simulink model "Wind_Turbine"  (R2025a)
settings: Solver=ode23t  StartTime=0.0  StopTime=70  MaxStep=0.01  RelTol=1e-4  AbsTol=1e-4  EnableMultiTasking=on
PreLoadFcn:
  | warning off Simulink:Commands:LoadMdlParameterizedLink
PostLoadFcn:
  | warning off Simulink:blocks:MatchingGotoNotFound
  | warning off Simulink:blocks:MatchingFromNotFound
  | warning('off','Simulink:SL_OutputNotConnected');
  | warning off Simulink:Engine:SaveWithParameterizedLinks_Warning
  | warning off Simulink:Engine:SaveWithDisabledLinks_Warning
  | warning('off','Simulink:fixpoint:fxpParameterPrecisionLoss');
  | warning off Simulink:blocks:DTConversionUncessary
  | warning off ne_sli:simulator:input:FilteredInputs
  | warning off MATLAB:nearlySingularMatrix
  | 
  | warning off xPCTarget:modeloptions:StackIncrease
  | warning off xPCTarget:sampleTime:sampleTimeInvariance
  | warning off Simulink:blocks:TDelayFixedBuffer
  | 
  | Setup_WT_Configurations
StartFcn:
  | tic
StopFcn:
  | Elapsed_Sim_Time = toc;
  | disp(['Elapsed time is ' num2str(Elapsed_Sim_Time)]);
undefined symbols (not defined in the file): sigbuilder_block, WT_Params, X, Y, Z
libraries: sm_lib x6, Wind_Lib x4, Yaw_System_Lib x4, Generator_Lib x3, Pitch_System_Lib x3, Pitch_Controller_Lib x3, Main_Controller_Lib x2, Geartrain_Lib x2, Hub_Axis_Lib x2, nesl_utility x2, Blades_Lib x1, Tower x1
Description:
  | Copyright 2009-2025 The MathWorks, Inc. MathWorks, Inc.
settings Model: ExtModeTrigDuration=100  Creator=smiller  LastModifiedBy=smiller
settings SolverCC: AutoScaleAbsTol=off  MaxConsecutiveMinStep=5  AlgebraicLoopSolver=TrustRegion  PositivePriorityOrder=on
settings DataIOCC: SaveFinalState=on  SaveFormat=StructureWithTime  ReturnWorkspaceOutputs=off
settings OptimizationCC: BlockReduction=off  OptimizeBlockIOStorage=off  BufferReuse=off  ReuseModelBlockBuffer=off  GlobalBufferReuse=off  ExpressionFolding=off  ExpressionDepthLimit=2147483647.0  LocalBlockOutputs=off  ZeroExternalMemoryAtStartup=off  ZeroInternalMemoryAtStartup=off  OptimizeDataStoreBuffers=off  BusAssignmentInplaceUpdate=off
settings DebuggingCC: AlgebraicLoopMsg=error  ArtificialAlgebraicLoopMsg=none  UnderspecifiedInitializationDetection=Classic  MergeDetectMultiDrivingBlocksExec=none  Int32ToFloatConvMsg=none  UnnecessaryDatatypeConvMsg=warning  FcnCallInpInsideContextMsg=warning  UnconnectedInputMsg=warning  UnconnectedOutputMsg=warning  UnconnectedLineMsg=warning  AllowSymbolicDim=off  StateNameClashWarn=warning  PregeneratedLibrarySubsystemCodeDiagnostic=none  SFUnexpectedBacktrackingDiag=warning  SFNoUnconditionalDefaultTransitionDiag=warning  SFExecutionAtInitializationDiag=none  ArithmeticOperatorsInVariantConditions=warning
settings HardwareCC: TargetBitPerPointer=64.0  TargetBitPerSizeT=64.0  TargetBitPerPtrDiffT=64.0  TargetLongLongMode=on  TargetIntDivRoundTo=Zero  TargetEndianess=LittleEndian  TargetWordSize=64.0  TargetHWDeviceType=MATLAB Host
settings ModelReferenceCC: EnableRefExpFcnMdlSchedulingChecks=on  PropagateSignalLabelsOutOfModel=off
settings SFSimCC: SimUseLocalCustomCode=off  SimParseCustomCode=off  CustomCodeUndefinedFunction=UseInterfaceOnly
settings RTWCC: RTWUseLocalCustomCode=off  Toolchain=Simulink Real-Time Toolchain  BuildConfiguration=Faster Runs  TargetLang=C++  GPUComputeCapability=3.5  DLArmComputeVersion=19.05
settings CodeAppCC: StateflowObjectComments=on
settings GRTTargetCC: TargetLangStandard=C++03 (ISO)  CodeInterfacePackaging=C++ class
settings ConfigComp: CovMetricSettings=dw  CovSaveCumulativeToWorkspaceVar=on  CovSaveSingleToWorkspaceVar=on  CovExternalEMLEnable=off  CovSFcnEnable=off
settings SimscapeCC: ExplicitSolverDiagnosticOptions=none  SimscapeNormalizeSystem=off  SimscapeLogType=all  SimscapeLogName=simlog_Wind_Turbine  SimscapeLogLimitData=off
settings ConfigurationSet: Description=SimMechanics 2G
settings ExplorerConfigSet: InternalSimMechanicsExplorerSettings="<ExplorerConfiguration><canonicalview>default</canonicalview><TilePanel><TileInfo><Tiles Columns=\"2\" Count=\"3\" Rows=\"2\"><Column Left=\"2\" Weight=\"0.6616\"/><Column Left=\"1076\" Weight=\"0.3384\"/><Column Left=\"1628\"/><Row Top=\"2\" Weight=\"0.4995\"/><Row Top=\"507\" Weight=\"0.5005\"/><Row Top=\"1014\"/><Tile Height=\"1\" Width=\"1\" X=\"0\" Y=\"0\"/><Tile Height=\"1\" Width=\"1\" X=\"0\" Y=\"1\"/><Tile Height=\"2\" Width=\"1\" X=\"1\" Y=\"0\"/></Tiles></TileInfo><SceneInfo><SceneViewer><BGColor><R>0.80000001192092896</R><G>1</G><B>1</B></BGColor><Camera><Position><X>151.73049973570119</X><Y>118.34405364859263</Y><Z>134.40663706667596</Z></Position><Center><X>-10.795458452286731</X><Y>-8.3649508446642677</Y><Z>101.0263657071233</Z></Center><Up><X>-0.12932527544138767</X><Y>-0.094165770600414006</Y><Z>0.98712095549595125</Z></Up><Left>-10.158594940113018</Left><Right>10.158594940113018</Right><Bottom>-7.1278539082560997</Bottom><Top>7.1278539082560997</Top></Camera></SceneViewer><SceneViewer><BGColor><R>0.80000001192092896</R><G>1</G><B>1</B></BGColor><Camera><Position><X>3.5719318734898633</X><Y>-0.12848459366052295</Y><Z>225.51131574619058</Z></Position><Center><X>-2.4920494569662206</X><Y>-0.0648600322177105</Y><Z>66.260519833710546</Z></Center><Up><X>0.0026243051834802709</X><Y>-0.99999643177881292</Y><Z>-0.00049945164542893202</Z></Up><Left>-11.826399210226041</Left><Right>11.826399210226041</Right><Bottom>-5.4233487502515896</Bottom><Top>5.4233487502515896</Top></Camera></SceneViewer><SceneViewer><BGColor><R>0.80000001192092896</R><G>1</G><B>1</B></BGColor><Camera><Position><X>121.9852231624925</X><Y>91.296071561311123</Y><Z>95.392428744838412</Z></Position><Center><X>2.8343002263369788</X><Y>-1.5967499794196209</Y><Z>70.920706290818515</Z></Center><Up><X>-0.12932527544138767</X><Y>-0.094165770600414006</Y><Z>0.98712095549595125</Z></Up><Left>-36.268603134155278</Left><Right>36.268603134155278</Right><Bottom>-73.406224822998055</Bottom><Top>73.406224822998055</Top></Camera></SceneViewer></SceneInfo></TilePanel></ExplorerConfiguration>"

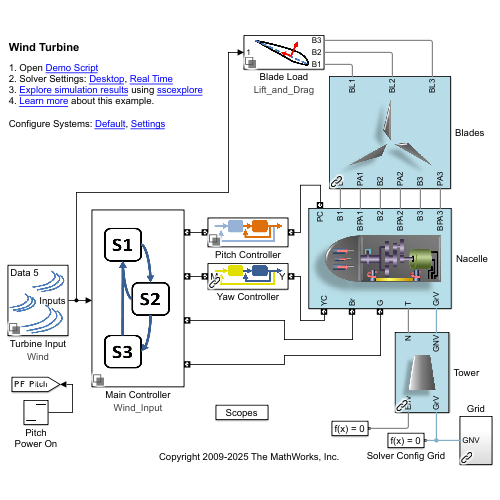
[thumbnail: Simulink's stored preview of the top-level diagram]
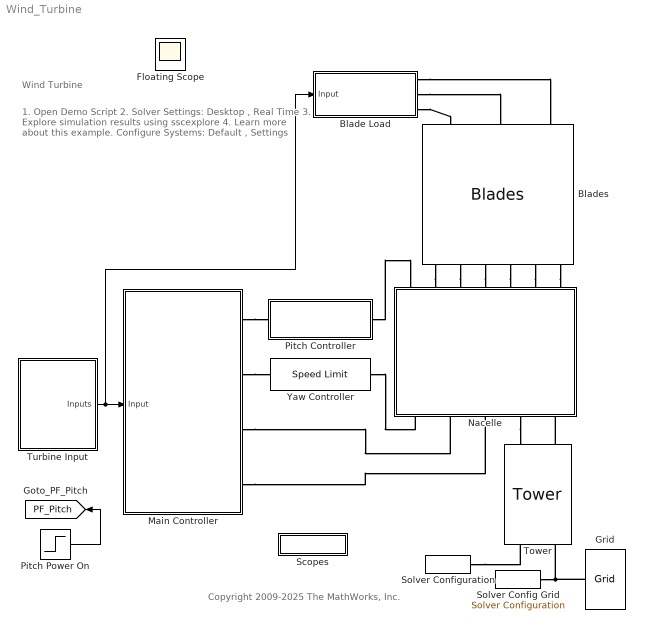
== system Wind_Turbine ==
  note: Copyright 2009-2025 The MathWorks, Inc.
  note: 1. Open Demo Script
      | 2. Solver Settings: Desktop , Real Time
      | 3. Explore simulation results using sscexplore
      | 4. Learn more about this example.
      |
      | Configure Systems: Default , Settings
  note: Wind Turbine
  Blade Load : Subsystem  Variant=on  VariantControlMode=label  LabelModeActiveChoice=Lift_and_Drag
      settings: AttributesFormatString=%<ActiveVariant>
      mask Display:
      | blk = wind_turbine_activeVariantBlock(gcb);
      | eval(get_param(blk, 'MaskDisplay'));
  Blades : Blades_Lib/Blades  RequirementInfo={} %GIDa_b4b772d6_2a4e_4d26_8c7e_f4f3f2f69a80  SystemSampleTime=-1  VariantActivationTime=update diagram  EmptyChoice=off  PassThrough=off  PassThroughVariantControl=(default)  EmptyChoiceVariantControl=(default)  AllowFlexibleInterface=on  Latency=0  AutoFrameSizeCalculation=off
  Grid : Generator_Lib/Grid  SystemSampleTime=-1  VariantActivationTime=update diagram  EmptyChoice=off  PassThrough=off  PassThroughVariantControl=(default)  EmptyChoiceVariantControl=(default)  AllowFlexibleInterface=on  Latency=0  AutoFrameSizeCalculation=off
  Main Controller : Subsystem  RequirementInfo={} %GIDa_306d441f_b8e1_436d_a194_501ebadfbc9d  Variant=on  VariantControlMode=label  LabelModeActiveChoice=Wind_Input
      settings: AttributesFormatString=%<ActiveVariant>
      mask Display:
      | blk = wind_turbine_activeVariantBlock(gcb);
      | eval(get_param(blk, 'MaskDisplay'));
  Nacelle : Subsystem
      mask Display:
      | PiA_Char = get_param([bdroot '/Nacelle/Pitch System'],'ActiveVariant');
      | YaA_Char = get_param([bdroot '/Nacelle/Yaw System'],'ActiveVariant');
      | Hub_Char = get_param([bdroot '/Nacelle/Hub Axis'],'ActiveVariant');
      | Gea_Char = get_param([bdroot '/Nacelle/Geartrain'],'ActiveVariant');
      | Gen_Char = get_param([bdroot '/Nacelle/Generator'],'ActiveVariant');
      | 
      | if(length(YaA_Char)<7)
      |     YaA_Char = 'LockedL';
      | end
      | 
      | image_str = ['Pi' PiA_Char(1) 'Ya' upper(YaA_Char(7)) 'Hu' Hub_Char(1) 'Ge' Gea_Char(1) 'Gn' Gen_Char(1)];
      | try
      |     image(['Nacelle_' image_str '_IMAGE.jpg']);
      | catch
      |     image('Nacelle_IMAGE.jpg');
      | end
  Pitch Power On : Step  Time=20  Before=24  After=24  SampleTime=0
  Pitch Controller : Subsystem  Variant=on  VariantControlMode=label  LabelModeActiveChoice=PI_on_AoA
      settings: AttributesFormatString=%<ActiveVariant>
      mask Display:
      | blk = wind_turbine_activeVariantBlock(gcb);
      | eval(get_param(blk, 'MaskDisplay'));
  Scopes : Subsystem
      mask Display: disp('Scopes');
  Solver Configuration : nesl_utility/Solver Configuration  PhysicalDomain=network_engine_domain  SubClassName=solver  LeftPortType=input  RightPortType=generic  Tones=[]  Harmonics=[]  SimulateNoise=off  Profile=off  UseLocalSampling=off  EnableSwitchedLinearOptims=on  FrequencyDomain=off  UseCCode=off  RelTol=0.001  AbsTol=1e-06  MinStep=1e-09  ToWorkspace=off  RevertToSquareIcSolve=off  NumHomotopyIterations=100  PhasorMode=off  PhasorModeNumHarmonics=1  ConsistencySolver=NEWTON_FTOL  IndexReductionMethod=DerivativeReplacement  DoDC=off  ResidualTolerance=1e-9  ConsistencyTolSource=GLOBAL  ConsistencyAbsTol=0.001  ConsistencyRelTol=0.001  ConsistencyTolFactor=0.001  UseLocalSolver=off  LocalSolverChoice=NE_BACKWARD_EULER_ADVANCER  ResolveIndetEquations=on  FunctionEvalNumThread=1  LocalSolverSampleTime=0.01  DoFixedCost=off  MaxNonlinIter=3  MaxModeIter=2  ComputeImpulses=off  ImpulseIterations=2  LinearAlgebra=Sparse  LinearAlgebraNumThread=0  EquationFormulation=NE_TIME_EF  DelaysMemoryBudget=1024  AutomaticFiltering=on  FilteringTimeConstant=0.001  PartitionStorageMethod=AS_NEEDED  PartitionMemoryBudget=1024  PartitionMethod=FAST  MultibodyUseLocalSolver=off  MultibodyLocalSolverChoice=ODE1  MultibodyLocalSolverSampleTime=0.001
  Solver Config Grid : nesl_utility/Solver Configuration  PhysicalDomain=network_engine_domain  SubClassName=solver  LeftPortType=input  RightPortType=generic  Tones=[]  Harmonics=[]  SimulateNoise=off  Profile=off  UseLocalSampling=off  EnableSwitchedLinearOptims=on  FrequencyDomain=off  UseCCode=off  RelTol=0.001  AbsTol=0.001  MinStep=1e-09  ToWorkspace=off  RevertToSquareIcSolve=off  NumHomotopyIterations=100  PhasorMode=off  PhasorModeNumHarmonics=1  ConsistencySolver=NEWTON_XTOL_AFTER_FTOL  IndexReductionMethod=None  DoDC=off  ResidualTolerance=1e-09  ConsistencyTolSource=GLOBAL  ConsistencyAbsTol=0.001  ConsistencyRelTol=0.001  ConsistencyTolFactor=1  UseLocalSolver=off  LocalSolverChoice=NE_BACKWARD_EULER_ADVANCER  ResolveIndetEquations=off  FunctionEvalNumThread=1  LocalSolverSampleTime=5e-5  DoFixedCost=off  MaxNonlinIter=2  MaxModeIter=2  ComputeImpulses=off  ImpulseIterations=2  LinearAlgebra=auto  LinearAlgebraNumThread=0  EquationFormulation=NE_FREQUENCY_TIME_EF  DelaysMemoryBudget=1024  AutomaticFiltering=off  FilteringTimeConstant=0.001  PartitionStorageMethod=AS_NEEDED  PartitionMemoryBudget=1024  PartitionMethod=ROBUST  MultibodyUseLocalSolver=off  MultibodyLocalSolverChoice=ODE1  MultibodyLocalSolverSampleTime=0.001
  Tower : Tower/Tower  RequirementInfo={} %GIDa_4943b1c2_7ab1_472c_939d_e8be874b5a74  SystemSampleTime=-1  VariantActivationTime=update diagram  EmptyChoice=off  PassThrough=off  PassThroughVariantControl=(default)  EmptyChoiceVariantControl=(default)  AllowFlexibleInterface=on  Latency=0  AutoFrameSizeCalculation=off
  Turbine Input : Subsystem  Variant=on  VariantControlMode=label  LabelModeActiveChoice=Wind
      settings: AttributesFormatString=%<ActiveVariant>
      mask Display:
      | blk = wind_turbine_activeVariantBlock(gcb);
      | eval(get_param(blk, 'MaskDisplay'));
      | 
      | 
      | if strcmp(get_param(gcb,'activevariant'),'Wind')
      |     [gr_ind, l] = signalbuilder([gcb '/Wind/Wind Input'], 'activegroup');
      |     text(0.05,0.9,['Data ' num2str(gr_ind)]);
      | end
  Yaw Controller : Yaw_Controller_Lib/Speed Limit  SystemSampleTime=-1  VariantActivationTime=update diagram  EmptyChoice=off  PassThrough=off  PassThroughVariantControl=(default)  EmptyChoiceVariantControl=(default)  AllowFlexibleInterface=on  Latency=0  AutoFrameSizeCalculation=off
  Floating Scope : Scope
  tag scope: PF_Pitch=global
  wires:
  Pitch Power On/1 -> [PF_Pitch]
  Turbine Input/1(Inputs) -> Main Controller/1(Input), Blade Load/1(Input)
  connections:
  Blades/LConn1 -- Nacelle/LConn2
  Pitch Controller/RConn1 -- Nacelle/LConn1
  Main Controller/RConn1 -- Pitch Controller/LConn1
  Nacelle/RConn4 -- Tower/LConn1
  Solver Configuration/RConn1 -- Tower/RConn1
  Blades/LConn5 -- Nacelle/LConn6
  Blades/LConn4 -- Nacelle/LConn5
  Blades/LConn3 -- Nacelle/LConn4
  Blades/LConn2 -- Nacelle/LConn3
  Blades/LConn6 -- Nacelle/LConn7
  Main Controller/RConn2 -- Yaw Controller/LConn1
  Main Controller/RConn4 -- Nacelle/RConn3
  Main Controller/RConn3 -- Nacelle/RConn2
  Blade Load/RConn3 -- Blades/RConn1
  Blade Load/RConn2 -- Blades/RConn2
  Blade Load/RConn1 -- Blades/RConn3
  Yaw Controller/RConn1 -- Nacelle/RConn1
  Solver Config Grid/RConn1 -- Grid/RConn1 -- Tower/RConn2
  Tower/LConn2 -- Nacelle/RConn5

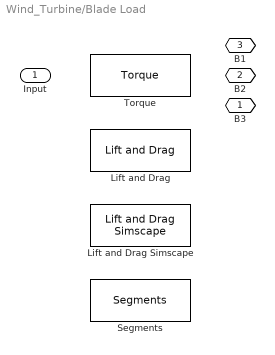
== system Wind_Turbine/Blade Load ==
  Input : Inport
  Lift and Drag : Wind_Lib/Lift and Drag  SystemSampleTime=-1  VariantControl=Lift_and_Drag  VariantActivationTime=update diagram  EmptyChoice=off  PassThrough=off  PassThroughVariantControl=(default)  EmptyChoiceVariantControl=(default)  AllowFlexibleInterface=on  Latency=0  AutoFrameSizeCalculation=off
  Lift and Drag Simscape : Wind_Lib/Lift and Drag Simscape  SystemSampleTime=-1  VariantControl=Lift_and_Drag_Simscape  VariantActivationTime=update diagram  EmptyChoice=off  PassThrough=off  PassThroughVariantControl=(default)  EmptyChoiceVariantControl=(default)  AllowFlexibleInterface=on  Latency=0  AutoFrameSizeCalculation=off
  Segments : Wind_Lib/Segments  SystemSampleTime=-1  VariantControl=Segments  VariantActivationTime=update diagram  EmptyChoice=off  PassThrough=off  PassThroughVariantControl=(default)  EmptyChoiceVariantControl=(default)  AllowFlexibleInterface=on  Latency=0  AutoFrameSizeCalculation=off
  Torque : Wind_Lib/Torque  SystemSampleTime=-1  VariantControl=Torque  VariantActivationTime=update diagram  EmptyChoice=off  PassThrough=off  PassThroughVariantControl=(default)  EmptyChoiceVariantControl=(default)  AllowFlexibleInterface=on  Latency=0  AutoFrameSizeCalculation=off
  B3 : PMIOPort  Side=Right
  B2 : PMIOPort  Port=2  Side=Right
  B1 : PMIOPort  Port=3  Side=Right

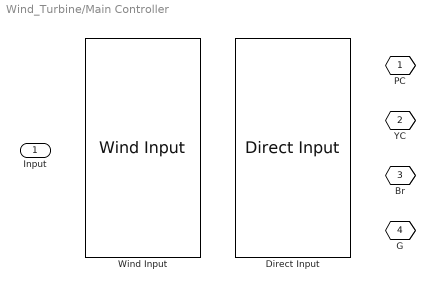
== system Wind_Turbine/Main Controller ==
  Input : Inport
  Direct Input : Main_Controller_Lib/Direct Input  SystemSampleTime=-1  VariantControl=Direct_Input  VariantActivationTime=update diagram  EmptyChoice=off  PassThrough=off  PassThroughVariantControl=(default)  EmptyChoiceVariantControl=(default)  AllowFlexibleInterface=on  Latency=0  AutoFrameSizeCalculation=off
  Wind Input : Main_Controller_Lib/Wind Input  SystemSampleTime=-1  VariantControl=Wind_Input  VariantActivationTime=update diagram  EmptyChoice=off  PassThrough=off  PassThroughVariantControl=(default)  EmptyChoiceVariantControl=(default)  AllowFlexibleInterface=on  Latency=0  AutoFrameSizeCalculation=off
  PC : PMIOPort  Tag=PMCPort  Side=Right
  YC : PMIOPort  Tag=PMCPort  Port=2  Side=Right
  Br : PMIOPort  Tag=PMCPort  Port=3  Side=Right
  G : PMIOPort  Tag=PMCPort  Port=4  Side=Right

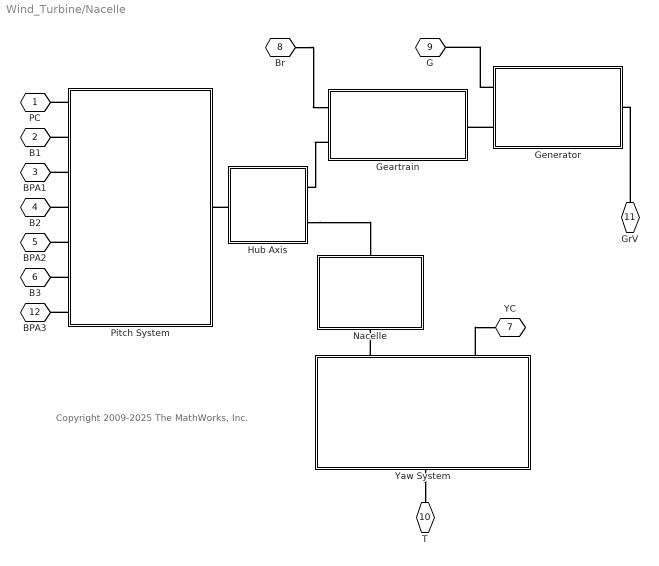
== system Wind_Turbine/Nacelle ==
  note: Copyright 2009-2025 The MathWorks, Inc.
  Geartrain : Subsystem  RequirementInfo={} %GIDa_0de6bbf9_bd2a_4f23_951e_791819310b87  Variant=on  VariantControlMode=label  LabelModeActiveChoice=Ideal
      settings: AttributesFormatString=%<ActiveVariant>
      mask Display:
      | blk = wind_turbine_activeVariantBlock(gcb);
      | eval(get_param(blk, 'MaskDisplay'));
  Generator : Subsystem  Variant=on  VariantControlMode=label  LabelModeActiveChoice=Full
      settings: AttributesFormatString=%<ActiveVariant>
      mask Display:
      | blk = wind_turbine_activeVariantBlock(gcb);
      | eval(get_param(blk, 'MaskDisplay'));
  Hub Axis : Subsystem  Tag=CustomStyle  Variant=on  VariantControlMode=label  LabelModeActiveChoice=Rotate
      settings: AttributesFormatString=%<ActiveVariant>
      mask Display:
      | blk = wind_turbine_activeVariantBlock(gcb);
      | eval(get_param(blk, 'MaskDisplay'));
  Nacelle : Subsystem
      mask Display:
      | image('Nacelle_Housing_IMAGE.jpg');
      | port_label('RConn',1,'N');
      | port_label('LConn',1,'YR');
  Pitch System : Subsystem  Tag=CustomStyle  RequirementInfo={} %GIDa_c1f640a7_49b6_45bd_a761_32e6bbcf8fa3  Variant=on  VariantControlMode=label  LabelModeActiveChoice=Ideal
      settings: AttributesFormatString=%<ActiveVariant>
      mask Display:
      | blk = wind_turbine_activeVariantBlock(gcb);
      | eval(get_param(blk, 'MaskDisplay'));
  Yaw System : Subsystem  Tag=CustomStyle  RequirementInfo={} %GIDa_39d3e21d_5d00_42ae_be4b_0d3d8be28763  Variant=on  VariantControlMode=label  LabelModeActiveChoice=Ideal_Actuator
      settings: AttributesFormatString=%<ActiveVariant>
      mask Display:
      | blk = wind_turbine_activeVariantBlock(gcb);
      | eval(get_param(blk, 'MaskDisplay'));
  PC : PMIOPort  Tag=PMCPort  Side=Left
  B1 : PMIOPort  Tag=PMCPort  Port=2  Side=Left
  BPA1 : PMIOPort  Tag=PMCPort  Port=3  Side=Left
  B2 : PMIOPort  Tag=PMCPort  Port=4  Side=Left
  BPA2 : PMIOPort  Tag=PMCPort  Port=5  Side=Left
  B3 : PMIOPort  Tag=PMCPort  Port=6  Side=Left
  YC : PMIOPort  Tag=PMCPort  Port=7  Side=Right
  Br : PMIOPort  Tag=PMCPort  Port=8  Side=Right
  G : PMIOPort  Tag=PMCPort  Port=9  Side=Right
  T : PMIOPort  Tag=PMCPort  Port=10  Side=Right
  GrV : PMIOPort  Tag=PMCPort  Port=11  Side=Right
  BPA3 : PMIOPort  Tag=PMCPort  Port=12  Side=Left
  connections:
  Hub Axis/LConn1 -- Pitch System/RConn1
  Yaw System/RConn1 -- Nacelle/LConn1
  Yaw System/LConn1 -- T/RConn1
  Br/RConn1 -- Geartrain/LConn1
  Pitch System/LConn7 -- BPA3/RConn1
  Pitch System/LConn5 -- BPA2/RConn1
  Pitch System/LConn3 -- BPA1/RConn1
  Pitch System/LConn6 -- B3/RConn1
  Generator/LConn2 -- Geartrain/RConn1
  Generator/LConn1 -- G/RConn1
  Pitch System/LConn1 -- PC/RConn1
  Pitch System/LConn4 -- B2/RConn1
  Pitch System/LConn2 -- B1/RConn1
  Hub Axis/RConn2 -- Nacelle/RConn1
  Yaw System/RConn2 -- YC/RConn1
  Geartrain/LConn2 -- Hub Axis/RConn1
  GrV/RConn1 -- Generator/RConn1

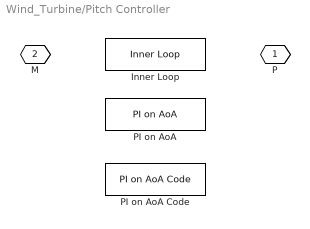
== system Wind_Turbine/Pitch Controller ==
  Inner Loop : Pitch_Controller_Lib/Inner Loop  SystemSampleTime=-1  VariantControl=Inner_Loop  VariantActivationTime=update diagram  EmptyChoice=off  PassThrough=off  PassThroughVariantControl=(default)  EmptyChoiceVariantControl=(default)  AllowFlexibleInterface=on  Latency=0  AutoFrameSizeCalculation=off
  PI on AoA : Pitch_Controller_Lib/PI on AoA  SystemSampleTime=-1  VariantControl=PI_on_AoA  VariantActivationTime=update diagram  EmptyChoice=off  PassThrough=off  PassThroughVariantControl=(default)  EmptyChoiceVariantControl=(default)  AllowFlexibleInterface=on  Latency=0  AutoFrameSizeCalculation=off
  PI on AoA Code : Pitch_Controller_Lib/PI on AoA Code  SystemSampleTime=-1  VariantControl=PI_on_AoA_Code  VariantActivationTime=update diagram  EmptyChoice=off  PassThrough=off  PassThroughVariantControl=(default)  EmptyChoiceVariantControl=(default)  AllowFlexibleInterface=on  Latency=0  AutoFrameSizeCalculation=off
  P : PMIOPort  Tag=PMCPort  Side=Right
  M : PMIOPort  Tag=PMCPort  Port=2  Side=Left

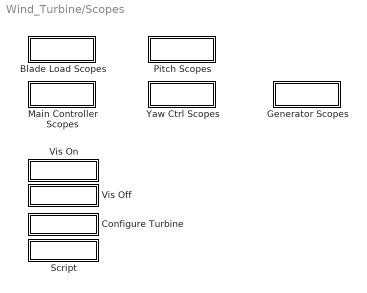
== system Wind_Turbine/Scopes ==
  Blade Load Scopes : Subsystem  ReferencedSubsystem=Blade_Load_Scopes
  Configure Turbine : Subsystem
      mask Display: disp('Configs');
  Generator Scopes : Subsystem  ReferencedSubsystem=Generator_Scopes
  Main Controller Scopes : Subsystem  ReferencedSubsystem=Main_Controller_Scopes
  Pitch Scopes : Subsystem  ReferencedSubsystem=Pitch_Scopes
  Script : Subsystem
      settings: OpenFcn=open('Wind_Turbine_Demo_Script.html')
      mask Display: disp('Script')
  Vis Off : Subsystem
      settings: OpenFcn=set_param(bdroot,'SimMechanicsOpenEditorOnUpdate','off');
      mask Display: disp('Vis Off')
  Vis On : Subsystem
      settings: OpenFcn=set_param(bdroot,'SimMechanicsOpenEditorOnUpdate','on');
      mask Display: disp('Vis On')
  Yaw Ctrl Scopes : Subsystem  ReferencedSubsystem=Yaw_Scopes

== system Wind_Turbine/Turbine Input ==
  Commands : Subsystem  VariantControl=Commands
      mask Display:
      | image(imread('Turbine_Input_Commands_IMAGE.jpg'));
      | port_label('output',1,'Inputs');
  Wind : Subsystem  VariantControl=Wind
      mask Display:
      | image('Turbine_Input_Wind_IMAGE.jpg');
      | port_label('output',1,'Inputs');
  Inputs : Outport  VectorParamsAs1DForOutWhenUnconnected=off

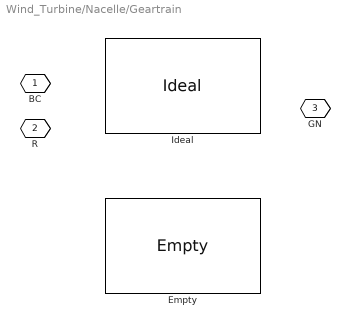
== system Wind_Turbine/Nacelle/Geartrain ==
  Empty : Geartrain_Lib/Empty  SystemSampleTime=-1  VariantControl=Empty  VariantActivationTime=update diagram  EmptyChoice=off  PassThrough=off  PassThroughVariantControl=(default)  EmptyChoiceVariantControl=(default)  AllowFlexibleInterface=on  Latency=0  AutoFrameSizeCalculation=off
  Ideal : Geartrain_Lib/Ideal  SystemSampleTime=-1  VariantControl=Ideal  VariantActivationTime=update diagram  EmptyChoice=off  PassThrough=off  PassThroughVariantControl=(default)  EmptyChoiceVariantControl=(default)  AllowFlexibleInterface=on  Latency=0  AutoFrameSizeCalculation=off
  BC : PMIOPort  Tag=PMCPort  Side=Left
  R : PMIOPort  Tag=PMCPort  Port=2  Side=Left
  GN : PMIOPort  Tag=PMCPort  Port=3  Side=Right

== system Wind_Turbine/Nacelle/Generator ==
  Full : Generator_Lib/Full  SystemSampleTime=-1  VariantControl=Full  VariantActivationTime=update diagram  EmptyChoice=off  PassThrough=off  PassThroughVariantControl=(default)  EmptyChoiceVariantControl=(default)  AllowFlexibleInterface=on  Latency=0  AutoFrameSizeCalculation=off
  Simple : Generator_Lib/Simple  SystemSampleTime=-1  VariantControl=Simple  VariantActivationTime=update diagram  EmptyChoice=off  PassThrough=off  PassThroughVariantControl=(default)  EmptyChoiceVariantControl=(default)  AllowFlexibleInterface=on  Latency=0  AutoFrameSizeCalculation=off
  M : PMIOPort  Tag=PMCPort  Side=Left
  G : PMIOPort  Port=2  Side=Left
  GrV : PMIOPort  Port=3  Side=Right

== system Wind_Turbine/Nacelle/Hub Axis ==
  Locked : Hub_Axis_Lib/Locked  SystemSampleTime=-1  VariantControl=Locked  VariantActivationTime=update diagram  EmptyChoice=off  PassThrough=off  PassThroughVariantControl=(default)  EmptyChoiceVariantControl=(default)  AllowFlexibleInterface=on  Latency=0  AutoFrameSizeCalculation=off
  Rotate : Hub_Axis_Lib/Rotate  SystemSampleTime=-1  VariantControl=Rotate  VariantActivationTime=update diagram  EmptyChoice=off  PassThrough=off  PassThroughVariantControl=(default)  EmptyChoiceVariantControl=(default)  AllowFlexibleInterface=on  Latency=0  AutoFrameSizeCalculation=off
  G : PMIOPort  Side=Right
  R : PMIOPort  Port=2  Side=Left
  N : PMIOPort  Port=3  Side=Right

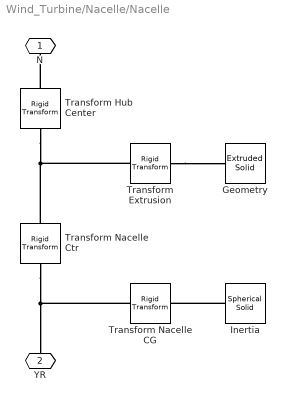
== system Wind_Turbine/Nacelle/Nacelle ==
  Geometry : sm_lib/Body Elements/Extruded Solid  ExtrusionType=General  PolygonNumSides=3  PolygonOuterRadius=1  PolygonOuterRadiusUnits=m  ExportEntireGeometry=off  ExtrusionCrossSection=WT_Params.Nacelle.Geometry.profile  ExtrusionCrossSectionUnits=m  ExportConvexHullGeometry=off  ExtrusionLength=WT_Params.Nacelle.length  ExtrusionLengthUnits=m  InertiaType=PointMass  BasedOnType=Density  Density=1000  DensityUnits=kg/(m^3)  Mass=0.1  MassUnits=kg  CenterOfMass=[0 0 0]  CenterOfMassUnits=m  MomentsOfInertia=[1 1 1]  MomentsOfInertiaUnits=kg*m^2  ProductsOfInertia=[0 0 0]  ProductsOfInertiaUnits=kg*m^2  GraphicType=FromGeometry  MarkerShape=Sphere  MarkerSize=10  GraphicVisPropType=SimpleVisualProperties  GraphicDiffuseColor=[0.8 0.8 0.8]  GraphicOpacity=1.0  GraphicSpecularColor=[0.5 0.5 0.5 1.0]  GraphicAmbientColor=[0.15 0.15 0.15 1.0]  GraphicEmissiveColor=[0.0 0.0 0.0 1.0]  GraphicShininess=75  DoExposeReferenceFrame=on  SerializedFrames=<Frames/>
  Inertia : sm_lib/Body Elements/Spherical Solid  SphereRadius=0.1  SphereRadiusUnits=m  ExportEntireGeometry=off  InertiaType=Custom  BasedOnType=Density  Density=1000  DensityUnits=kg/(m^3)  Mass=WT_Params.Nacelle.mass  MassUnits=kg  CenterOfMass=[0 0 0]  CenterOfMassUnits=m  MomentsOfInertia=[WT_Params.Nacelle.inertia(1,1) WT_Params.Nacelle.inertia(3,3) WT_Params.Nacelle.inertia(2,2)]  MomentsOfInertiaUnits=kg*m^2  ProductsOfInertia=[0 0 0]  ProductsOfInertiaUnits=kg*m^2  GraphicType=FromGeometry  MarkerShape=Sphere  MarkerSize=10  GraphicVisPropType=SimpleVisualProperties  GraphicDiffuseColor=[0.8 0.8 0.8]  GraphicOpacity=1.0  GraphicSpecularColor=[0.5 0.5 0.5 1.0]  GraphicAmbientColor=[0.15 0.15 0.15 1.0]  GraphicEmissiveColor=[0.0 0.0 0.0 1.0]  GraphicShininess=75  DoExposeReferenceFrame=on  SerializedFrames=<Frames/>
  Transform Extrusion : sm_lib/Frames and Transforms/Rigid Transform  RotationMethod=StandardAxis  FollAlignAxisA=+X  BaseAlignAxisA=+Y  FollAlignAxisB=+Y  BaseAlignAxisB=+Z  RotationStandardAxis=+Y  RotationAngle=90  RotationAngleUnits=deg  RotationArbitraryAxis=[0 0 1]  RotationSequenceAxes=FollowerAxes  RotationSequence=XYX  RotationSequenceAngles=[0 0 0]  RotationSequenceAnglesUnits=deg  RotationMatrix=[1 0 0; 0 1 0; 0 0 1]  Quaternion=[1 0 0 0]  TranslationMethod=Cartesian  TranslationCartesianOffset=[0 0 0]  TranslationCartesianOffsetUnits=m  TranslationStandardAxis=+Z  TranslationStandardOffset=1  TranslationStandardOffsetUnits=m  TranslationROffset=0  TranslationROffsetUnits=m  TranslationThetaOffset=0  TranslationThetaOffsetUnits=deg  TranslationZOffset=0  TranslationZOffsetUnits=m
  Transform Hub Center : sm_lib/Frames and Transforms/Rigid Transform  RotationMethod=StandardAxis  FollAlignAxisA=+X  BaseAlignAxisA=+Y  FollAlignAxisB=+Y  BaseAlignAxisB=+Z  RotationStandardAxis=+Y  RotationAngle=90  RotationAngleUnits=deg  RotationArbitraryAxis=[0 0 1]  RotationSequenceAxes=FollowerAxes  RotationSequence=XYX  RotationSequenceAngles=[0 0 0]  RotationSequenceAnglesUnits=deg  RotationMatrix=[1 0 0; 0 1 0; 0 0 1]  Quaternion=[1 0 0 0]  TranslationMethod=StandardAxis  TranslationCartesianOffset=[0 0 0]  TranslationCartesianOffsetUnits=m  TranslationStandardAxis=+X  TranslationStandardOffset=WT_Params.Nacelle.length/2  TranslationStandardOffsetUnits=m  TranslationROffset=0  TranslationROffsetUnits=m  TranslationThetaOffset=0  TranslationThetaOffsetUnits=deg  TranslationZOffset=0  TranslationZOffsetUnits=m
  Transform Nacelle CG : sm_lib/Frames and Transforms/Rigid Transform  RotationMethod=None  FollAlignAxisA=+X  BaseAlignAxisA=+Y  FollAlignAxisB=+Y  BaseAlignAxisB=+Z  RotationStandardAxis=+Z  RotationAngle=0  RotationAngleUnits=deg  RotationArbitraryAxis=[0 0 1]  RotationSequenceAxes=FollowerAxes  RotationSequence=XYX  RotationSequenceAngles=[0 0 0]  RotationSequenceAnglesUnits=deg  RotationMatrix=[1 0 0; 0 1 0; 0 0 1]  Quaternion=[1 0 0 0]  TranslationMethod=Cartesian  TranslationCartesianOffset=[-WT_Params.Nacelle.Yaw_Ctr_Offset.x+WT_Params.Nacelle.CG_Offset.x 0 WT_Params.Nacelle.Yaw_Ctr_Offset.y]  TranslationCartesianOffsetUnits=m  TranslationStandardAxis=+Z  TranslationStandardOffset=1  TranslationStandardOffsetUnits=m  TranslationROffset=0  TranslationROffsetUnits=m  TranslationThetaOffset=0  TranslationThetaOffsetUnits=deg  TranslationZOffset=0  TranslationZOffsetUnits=m
  Transform Nacelle Ctr : sm_lib/Frames and Transforms/Rigid Transform  RotationMethod=None  FollAlignAxisA=+X  BaseAlignAxisA=+Y  FollAlignAxisB=+Y  BaseAlignAxisB=+Z  RotationStandardAxis=+Z  RotationAngle=0  RotationAngleUnits=deg  RotationArbitraryAxis=[0 0 1]  RotationSequenceAxes=FollowerAxes  RotationSequence=XYX  RotationSequenceAngles=[0 0 0]  RotationSequenceAnglesUnits=deg  RotationMatrix=[1 0 0; 0 1 0; 0 0 1]  Quaternion=[1 0 0 0]  TranslationMethod=Cartesian  TranslationCartesianOffset=[-WT_Params.Nacelle.length/2+3 0 WT_Params.Nacelle.Yaw_Ctr_Offset.y]  TranslationCartesianOffsetUnits=m  TranslationStandardAxis=+Z  TranslationStandardOffset=1  TranslationStandardOffsetUnits=m  TranslationROffset=0  TranslationROffsetUnits=m  TranslationThetaOffset=0  TranslationThetaOffsetUnits=deg  TranslationZOffset=0  TranslationZOffsetUnits=m
  N : PMIOPort  Side=Right
  YR : PMIOPort  Port=2  Side=Left
  connections:
  Transform Nacelle Ctr/LConn1 -- YR/RConn1 -- Transform Nacelle CG/LConn1
  Transform Nacelle Ctr/RConn1 -- Transform Extrusion/LConn1 -- Transform Hub Center/LConn1
  Transform Hub Center/RConn1 -- N/RConn1
  Inertia/RConn1 -- Transform Nacelle CG/RConn1
  Transform Extrusion/RConn1 -- Geometry/RConn1

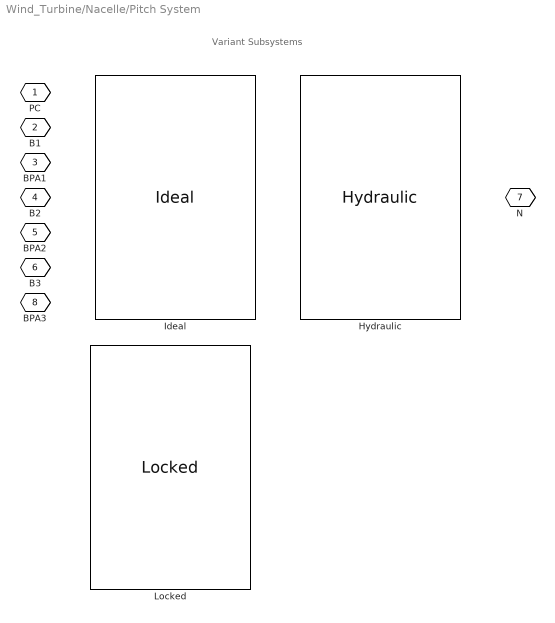
== system Wind_Turbine/Nacelle/Pitch System ==
  note: Variant Subsystems
  Hydraulic : Pitch_System_Lib/Hydraulic  SystemSampleTime=-1  VariantControl=Hydraulic  VariantActivationTime=update diagram  EmptyChoice=off  PassThrough=off  PassThroughVariantControl=(default)  EmptyChoiceVariantControl=(default)  AllowFlexibleInterface=on  Latency=0  AutoFrameSizeCalculation=off
  Ideal : Pitch_System_Lib/Ideal  SystemSampleTime=-1  VariantControl=Ideal  VariantActivationTime=update diagram  EmptyChoice=off  PassThrough=off  PassThroughVariantControl=(default)  EmptyChoiceVariantControl=(default)  AllowFlexibleInterface=on  Latency=0  AutoFrameSizeCalculation=off
  Locked : Pitch_System_Lib/Locked  SystemSampleTime=-1  VariantControl=Locked  VariantActivationTime=update diagram  EmptyChoice=off  PassThrough=off  PassThroughVariantControl=(default)  EmptyChoiceVariantControl=(default)  AllowFlexibleInterface=on  Latency=0  AutoFrameSizeCalculation=off
  PC : PMIOPort  Tag=PMCPort  Side=Left
  B1 : PMIOPort  Tag=PMCPort  Port=2  Side=Left
  BPA1 : PMIOPort  Tag=PMCPort  Port=3  Side=Left
  B2 : PMIOPort  Tag=PMCPort  Port=4  Side=Left
  BPA2 : PMIOPort  Tag=PMCPort  Port=5  Side=Left
  B3 : PMIOPort  Tag=PMCPort  Port=6  Side=Left
  N : PMIOPort  Tag=PMCPort  Port=7  Side=Right
  BPA3 : PMIOPort  Tag=PMCPort  Port=8  Side=Left

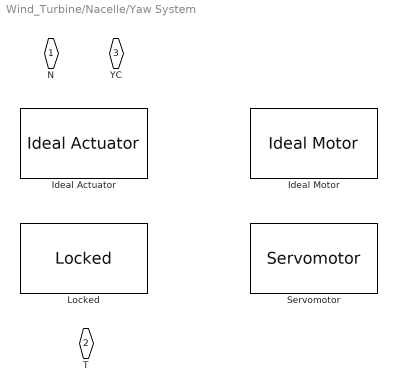
== system Wind_Turbine/Nacelle/Yaw System ==
  Ideal Actuator : Yaw_System_Lib/Ideal Actuator  SystemSampleTime=-1  VariantControl=Ideal_Actuator  VariantActivationTime=update diagram  EmptyChoice=off  PassThrough=off  PassThroughVariantControl=(default)  EmptyChoiceVariantControl=(default)  AllowFlexibleInterface=on  Latency=0  AutoFrameSizeCalculation=off
  Ideal Motor : Yaw_System_Lib/Ideal Motor  SystemSampleTime=-1  VariantControl=Ideal_Motor  VariantActivationTime=update diagram  EmptyChoice=off  PassThrough=off  PassThroughVariantControl=(default)  EmptyChoiceVariantControl=(default)  AllowFlexibleInterface=on  Latency=0  AutoFrameSizeCalculation=off
  Locked : Yaw_System_Lib/Locked  SystemSampleTime=-1  VariantControl=Locked  VariantActivationTime=update diagram  EmptyChoice=off  PassThrough=off  PassThroughVariantControl=(default)  EmptyChoiceVariantControl=(default)  AllowFlexibleInterface=on  Latency=0  AutoFrameSizeCalculation=off
  Servomotor : Yaw_System_Lib/Servomotor  SystemSampleTime=-1  VariantControl=Servomotor  VariantActivationTime=update diagram  EmptyChoice=off  PassThrough=off  PassThroughVariantControl=(default)  EmptyChoiceVariantControl=(default)  AllowFlexibleInterface=on  Latency=0  AutoFrameSizeCalculation=off
  N : PMIOPort  Side=Right
  T : PMIOPort  Port=2  Side=Left
  YC : PMIOPort  Port=3  Side=Right

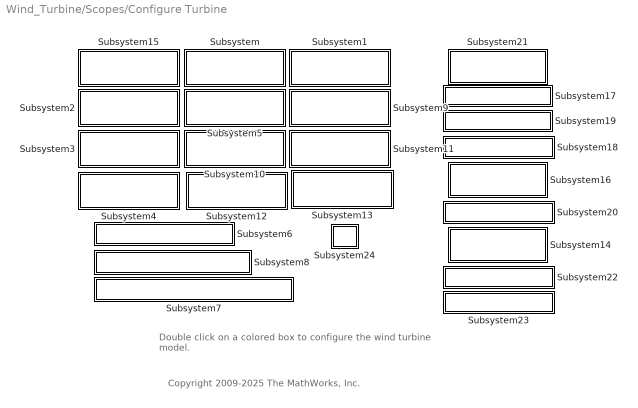
== system Wind_Turbine/Scopes/Configure Turbine ==
  note: Copyright 2009-2025 The MathWorks, Inc.
  note: Double click on a colored box
      | to configure the wind turbine model.
  Subsystem : Subsystem
      settings: OpenFcn=Select_Turbine_Systems('I_Pitch Test', WT_Configs)
      mask Display: disp('Ideal\nPitch')
  Subsystem1 : Subsystem
      settings: OpenFcn=Select_Turbine_Systems('H_Pitch Test', WT_Configs)
      mask Display: disp('Hydraulic\nPitch')
  Subsystem10 : Subsystem
      settings: OpenFcn=Select_Turbine_Systems('I_Pitch IM_Yaw Test', WT_Configs)
      mask Display: disp('Ideal Pitch\nIdeal Motor Yaw')
  Subsystem11 : Subsystem
      settings: OpenFcn=Select_Turbine_Systems('H_Pitch IM_Yaw Test', WT_Configs)
      mask Display: disp('Hydraulic Pitch\nIdeal Motor Yaw')
  Subsystem12 : Subsystem
      settings: OpenFcn=Select_Turbine_Systems('I_Pitch S_Yaw Test', WT_Configs)
      mask Display: disp('Ideal Pitch\nServomotor Yaw')
  Subsystem13 : Subsystem
      settings: OpenFcn=Select_Turbine_Systems('H_Pitch S_Yaw Test', WT_Configs)
      mask Display: disp('Hydraulic Pitch\nServomotor Yaw')
  Subsystem14 : Subsystem
      settings: OpenFcn=Compare_Yaw_Actuators;
      mask Display: disp('Compare Yaw\nActuators')
  Subsystem15 : Subsystem
      mask Display: disp('TESTS')
  Subsystem16 : Subsystem
      settings: OpenFcn=Compare_Pitch_Actuators;
      mask Display: disp('Compare Pitch\nActuators')
  Subsystem17 : Subsystem
      settings: OpenFcn=Pitch_Actuation_Linkage
      mask Display: disp('Pitch Linkage')
  Subsystem18 : Subsystem
      settings: OpenFcn=Pitch_Actuation_Hydraulic_Testrig
      mask Display: disp('Hydr. Pitch Testrig')
  Subsystem19 : Subsystem
      settings: OpenFcn=Pitch_Control_Ideal_Testrig
      mask Display: disp('Ideal Pitch Testrig')
  Subsystem2 : Subsystem
      settings: OpenFcn=Select_Turbine_Systems('IA_Yaw Test', WT_Configs)
      mask Display: disp('Ideal Actuator\nYaw')
  Subsystem20 : Subsystem
      settings: OpenFcn=Yaw_Actuation_Testrig
      mask Display: disp('Yaw Testrig')
  Subsystem21 : Subsystem
      mask Display: disp('DEVELOP')
  Subsystem22 : Subsystem
      settings: OpenFcn=Generator_Testrig
      mask Display: disp('Generator Testrig')
  Subsystem23 : Subsystem
      settings: OpenFcn=Turbine_State_Machine_Testrig
      mask Display: disp('Supervisory Ctrl')
  Subsystem24 : Subsystem
      settings: OpenFcn=Select_Turbine_Systems('H_Pitch S_Yaw Ge Gn Lift_Drag', WT_Configs)
      mask Display: disp('C')
  Subsystem3 : Subsystem
      settings: OpenFcn=Select_Turbine_Systems('IM_Yaw Test', WT_Configs)
      mask Display: disp('Ideal Motor\nYaw')
  Subsystem4 : Subsystem
      settings: OpenFcn=Select_Turbine_Systems('S_Yaw Test', WT_Configs)
      mask Display: disp('Servomotor\nYaw')
  Subsystem5 : Subsystem
      settings: OpenFcn=Select_Turbine_Systems('I_Pitch IA_Yaw Test', WT_Configs)
      mask Display: disp('Ideal Pitch\nIdeal Act. Yaw')
  Subsystem6 : Subsystem
      settings: OpenFcn=Select_Turbine_Systems('I_Pitch IA_Yaw Lift_Drag', WT_Configs)
      mask Display: disp('I Pitch IA Yaw Lift Drag')
  Subsystem7 : Subsystem
      settings: OpenFcn=Select_Turbine_Systems('I_Pitch IA_Yaw Ge Gn Lift_Drag', WT_Configs)
      mask Display: disp('I_Pitch IA_Yaw Ge Gn Lift_Drag')
  Subsystem8 : Subsystem
      settings: OpenFcn=Select_Turbine_Systems('I_Pitch IA_Yaw Ge Lift_Drag', WT_Configs)
      mask Display: disp('I Pitch IA Yaw Ge Lift Drag')
  Subsystem9 : Subsystem
      settings: OpenFcn=Select_Turbine_Systems('H_Pitch IA_Yaw Test', WT_Configs)
      mask Display: disp('Hydraulic Pitch\nIdeal Act. Yaw')

== system Wind_Turbine/Scopes/Script ==

== system Wind_Turbine/Scopes/Vis Off ==

== system Wind_Turbine/Scopes/Vis On ==

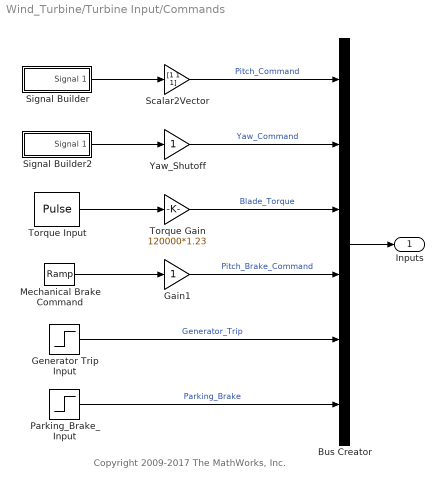
== system Wind_Turbine/Turbine Input/Commands ==
  note: Copyright 2009-2017 The MathWorks, Inc.
  Bus Creator : BusCreator  Inputs=6
  Gain1 : Gain
  Generator Trip Input : Step  Time=90  Before=1  SampleTime=0
  Mechanical Brake Command : simulink/Sources/Ramp  slope=1  start=40  InitialOutput=0
  Parking_Brake_Input : Step  Time=5  Before=1  After=0  SampleTime=0
  Scalar2Vector : Gain  Gain=[1 1 1]
  Signal Builder : Subsystem  Tag=STV Subsys  LoadFcn=sigbuilder_block('load');  StartFcn=sigbuilder_block('start');  StopFcn=sigbuilder_block('stop');  ClipboardFcn=sigbuilder_block('clipboard');  mask(Sigbuilder block){tuvar=[0:10]}
      mask help: Sigbuilder GUI
      mask init:
      | if ~strcmp(get_param(bdroot(gcbh),'SimulationStatus'),'stopped') tuvar = sigbuilder_block('maskInit'); end
      settings: CopyFcn=sigbuilder_block('copy');  DeleteFcn=sigbuilder_block('delete');  ModelCloseFcn=sigbuilder_block('modelClose');  PreSaveFcn=sigbuilder_block('preSave');  PauseFcn=sigbuilder_block('pause')  ContinueFcn=sigbuilder_block('continue')  NameChangeFcn=sigbuilder_block('namechange');  OpenFcn=sigbuilder_block('open',[214.5 254.25 550.5 399.75 ]);  CloseFcn=sigbuilder_block('close');
      mask Display: plot(0, 0, 100, 100,[2, 2, 32, 32, 2], [68, 8, 8, 68, 68],[32, 2], [38, 38], [32, 19, 2],[53, 60, 44], [32, 17, 17, 2],[16, 16, 31, 31]);txt = getActiveGroup(gcbh);text(2, 100, txt,'verticalAlignment', 'top');
  Signal Builder2 : Subsystem  Tag=STV Subsys  LoadFcn=sigbuilder_block('load');  StartFcn=sigbuilder_block('start');  StopFcn=sigbuilder_block('stop');  ClipboardFcn=sigbuilder_block('clipboard');  mask(Sigbuilder block){tuvar=[0:10]}
      mask help: Sigbuilder GUI
      mask init:
      | if ~strcmp(get_param(bdroot(gcbh),'SimulationStatus'),'stopped') tuvar = sigbuilder_block('maskInit'); end
      settings: CopyFcn=sigbuilder_block('copy');  DeleteFcn=sigbuilder_block('delete');  ModelCloseFcn=sigbuilder_block('modelClose');  PreSaveFcn=sigbuilder_block('preSave');  PauseFcn=sigbuilder_block('pause')  ContinueFcn=sigbuilder_block('continue')  NameChangeFcn=sigbuilder_block('namechange');  OpenFcn=sigbuilder_block('open',[28.5 161.25 550.5 489 ]);  CloseFcn=sigbuilder_block('close');
      mask Display: plot(0, 0, 100, 100,[2, 2, 32, 32, 2], [68, 8, 8, 68, 68],[32, 2], [38, 38], [32, 19, 2],[53, 60, 44], [32, 17, 17, 2],[16, 16, 31, 31]);txt = getActiveGroup(gcbh);text(2, 100, txt,'verticalAlignment', 'top');
  Torque Gain : Gain  Gain=120000*1.23
  Torque Input : DiscretePulseGenerator  PulseType=Time based  Amplitude=10  Period=100  PulseWidth=10
  Yaw_Shutoff : Gain
  Inputs : Outport  VectorParamsAs1DForOutWhenUnconnected=off
  wires:
  Bus Creator/1 -> Inputs/1
  Signal Builder2/1(Signal 1) -> Yaw_Shutoff/1
  Signal Builder/1(Signal 1) -> Scalar2Vector/1
  Torque Input/1 -> Torque Gain/1
  Scalar2Vector/1 -> Bus Creator/1  "Pitch_Command"
  Yaw_Shutoff/1 -> Bus Creator/2  "Yaw_Command"
  Torque Gain/1 -> Bus Creator/3  "Blade_Torque"
  Mechanical Brake Command/1 -> Gain1/1
  Generator Trip Input/1 -> Bus Creator/5  "Generator_Trip"
  Gain1/1 -> Bus Creator/4  "Pitch_Brake_Command"
  Parking_Brake_Input/1 -> Bus Creator/6  "Parking_Brake"

== system Wind_Turbine/Turbine Input/Wind ==
  Mux1 : Mux  Inputs=2
  Wind Input : Subsystem  Tag=STV Subsys  LoadFcn=sigbuilder_block('load');  StartFcn=sigbuilder_block('start');  StopFcn=sigbuilder_block('stop');  ClipboardFcn=sigbuilder_block('clipboard');  mask(Sigbuilder block){tuvar=[0:10]}
      mask help: Sigbuilder GUI
      mask init:
      | if ~strcmp(get_param(bdroot(gcbh),'SimulationStatus'),'stopped') tuvar = sigbuilder_block('maskInit'); end
      settings: CopyFcn=sigbuilder_block('copy');  DeleteFcn=sigbuilder_block('delete');  ModelCloseFcn=sigbuilder_block('modelClose');  PreSaveFcn=sigbuilder_block('preSave');  PauseFcn=sigbuilder_block('pause')  ContinueFcn=sigbuilder_block('continue')  NameChangeFcn=sigbuilder_block('namechange');  OpenFcn=sigbuilder_block('open',[17.4 220.2 762 360.6 ]);  CloseFcn=sigbuilder_block('close');
      mask Display: plot(0, 0, 100, 100,[2, 2, 32, 32, 2], [68, 8, 8, 68, 68],[32, 2], [38, 38], [32, 19, 2],[53, 60, 44], [32, 17, 17, 2],[16, 16, 31, 31]);txt = getActiveGroup(gcbh);text(2, 100, txt,'verticalAlignment', 'top');
  Inputs : Outport  VectorParamsAs1DForOutWhenUnconnected=off
  wires:
  Mux1/1 -> Inputs/1
  Wind Input/1(Wind Speed) -> Mux1/1
  Wind Input/2(Wind Direction) -> Mux1/2

== system Wind_Turbine/Scopes/Configure Turbine/Subsystem ==

== system Wind_Turbine/Scopes/Configure Turbine/Subsystem1 ==

== system Wind_Turbine/Scopes/Configure Turbine/Subsystem10 ==

== system Wind_Turbine/Scopes/Configure Turbine/Subsystem11 ==

== system Wind_Turbine/Scopes/Configure Turbine/Subsystem12 ==

== system Wind_Turbine/Scopes/Configure Turbine/Subsystem13 ==

== system Wind_Turbine/Scopes/Configure Turbine/Subsystem14 ==

== system Wind_Turbine/Scopes/Configure Turbine/Subsystem15 ==

== system Wind_Turbine/Scopes/Configure Turbine/Subsystem16 ==

== system Wind_Turbine/Scopes/Configure Turbine/Subsystem17 ==

== system Wind_Turbine/Scopes/Configure Turbine/Subsystem18 ==

== system Wind_Turbine/Scopes/Configure Turbine/Subsystem19 ==

== system Wind_Turbine/Scopes/Configure Turbine/Subsystem2 ==

== system Wind_Turbine/Scopes/Configure Turbine/Subsystem20 ==

== system Wind_Turbine/Scopes/Configure Turbine/Subsystem21 ==

== system Wind_Turbine/Scopes/Configure Turbine/Subsystem22 ==

== system Wind_Turbine/Scopes/Configure Turbine/Subsystem23 ==

== system Wind_Turbine/Scopes/Configure Turbine/Subsystem24 ==

== system Wind_Turbine/Scopes/Configure Turbine/Subsystem3 ==

== system Wind_Turbine/Scopes/Configure Turbine/Subsystem4 ==

== system Wind_Turbine/Scopes/Configure Turbine/Subsystem5 ==

== system Wind_Turbine/Scopes/Configure Turbine/Subsystem6 ==

== system Wind_Turbine/Scopes/Configure Turbine/Subsystem7 ==

== system Wind_Turbine/Scopes/Configure Turbine/Subsystem8 ==

== system Wind_Turbine/Scopes/Configure Turbine/Subsystem9 ==

== system Wind_Turbine/Turbine Input/Commands/Signal Builder ==
  Demux : Demux  Tag=STV Demux  Outputs=1
      settings: DisplayOption=none
  FromWs : FromWorkspace  Tag=STV FromWs  VariableName=tuvar
      SigBuilderData=|
      | common.afterFinalStr = 'Extrapolate'
      | common.sampleTime = 0
      | dataSet(1).timeRange = [0 50]
      | dataSet(1).name = 'Pos_Test'
      | dataSet(2).timeRange = [0 50]
      | dataSet(2).name = 'Pos_Neg_Test'
      | dataSet(3).timeRange = [0 50]
      | dataSet(3).name = 'Step_Test'
      | sbobj.Groups(1).Name = 'Pos_Test'
      | sbobj.Groups(1).Signals.Name = 'Signal 1'
      | sbobj.Groups(1).Signals.XData = [0 5 5 7.5 7.5 25.1 25.1 28 28 50]
      | sbobj.Groups(1).Signals.YData = [0 0 20 20 0 0 20 20 0 0]
      | sbobj.Groups(1).TimeRange = [0 50]
      | sbobj.Groups(2).Name = 'Pos_Neg_Test'
      | sbobj.Groups(2).Signals.Name = 'Signal 1'
      | sbobj.Groups(2).Signals.XData = [0 3 3 5.5 5.5 8 8 10.5 10.5 50]
      | sbobj.Groups(2).Signals.YData = [0 0 20 20 0 0 -20 -20 0 0]
      | sbobj.Groups(2).TimeRange = [0 50]
      | sbobj.Groups(3).Name = 'Step_Test'
      | sbobj.Groups(3).Signals.Name = 'Signal 1'
      | sbobj.Groups(3).Signals.XData = [0 1 1 7.5 25.1 30 30 50]
      | sbobj.Groups(3).Signals.YData = [0 0 20 20 20 20 0 0]
      | sbobj.Groups(3).TimeRange = [0 50]
  Signal 1 : Outport  Tag=STV Outport  VectorParamsAs1DForOutWhenUnconnected=off
  wires:
  Demux/1 -> Signal 1/1
  FromWs/1 -> Demux/1

== system Wind_Turbine/Turbine Input/Commands/Signal Builder2 ==
  Demux : Demux  Tag=STV Demux  Outputs=1
      settings: DisplayOption=none
  FromWs : FromWorkspace  Tag=STV FromWs  VariableName=tuvar
      SigBuilderData=|
      | common.afterFinalStr = 'Extrapolate'
      | common.sampleTime = 0
      | dataSet(1).timeRange = [0 50]
      | dataSet(1).name = 'Pos_Neg_Test'
      | dataSet(2).timeRange = [0 50]
      | dataSet(2).name = 'Step_Test'
      | dataSet(3).timeRange = [0 50]
      | dataSet(3).name = 'Ramp_Test'
      | sbobj.Groups(1).Name = 'Pos_Neg_Test'
      | sbobj.Groups(1).Signals.Name = 'Signal 1'
      | sbobj.Groups(1).Signals.XData = [0 1 1 11 11 21 21 31 31 50]
      | sbobj.Groups(1).Signals.YData = [0 0 4 4 0 0 -4 -4 0 0]
      | sbobj.Groups(2).Name = 'Step_Test'
      | sbobj.Groups(2).Signals.Name = 'Signal 1'
      | sbobj.Groups(2).Signals.XData = [0 1 1 11 21 31 31 50]
      | sbobj.Groups(2).Signals.YData = [0 0 4 4 4 4 0 0]
      | sbobj.Groups(3).Name = 'Ramp_Test'
      | sbobj.Groups(3).Signals.Name = 'Signal 1'
      | sbobj.Groups(3).Signals.XData = [0 1 1 11 21 31 39.1 50]
      | sbobj.Groups(3).Signals.YData = [0 0 2.46 4 2.32 3.18 1.16 0]
  Signal 1 : Outport  Tag=STV Outport  VectorParamsAs1DForOutWhenUnconnected=off
  wires:
  Demux/1 -> Signal 1/1
  FromWs/1 -> Demux/1

== system Wind_Turbine/Turbine Input/Wind/Wind Input ==
  Demux : Demux  Tag=STV Demux  Outputs=2
      settings: DisplayOption=none
  FromWs : FromWorkspace  Tag=STV FromWs  VariableName=tuvar
      SigBuilderData=|
      | common.afterFinalStr = 'Extrapolate'
      | common.sampleTime = 0
      | dataSet(1).timeRange = [0 130]
      | dataSet(1).name = 'Constant Wind No Yaw'
      | dataSet(2).timeRange = [0 130]
      | dataSet(2).name = 'Constant Wind'
      | dataSet(3).timeRange = [0 60]
      | dataSet(3).name = 'High Wind Speed'
      | dataSet(4).timeRange = [0 130]
      | dataSet(4).name = 'Cut Out'
      | dataSet(5).timeRange = [0 130]
      | dataSet(5).name = 'Start Stop'
      | dataSet(6).timeRange = [0 130]
      | dataSet(6).name = 'Start Stop No Yaw'
      | dataSet(7).timeRange = [0 130]
      | dataSet(7).name = 'Varying Wind'
      | sbobj.Groups(1).Name = 'Constant Wind No Yaw'
      | sbobj.Groups(1).Signals(1).Name = 'Wind Speed'
      | sbobj.Groups(1).Signals(1).XData = [0 10 130]
      | sbobj.Groups(1).Signals(1).YData = [10 10 10]
      | sbobj.Groups(1).Signals(2).Name = 'Wind Direction'
      | sbobj.Groups(1).Signals(2).XData = [0 1 11 21 31 130]
      | sbobj.Groups(1).Signals(2).YData = [0 0 0 0 0 0]
      | sbobj.Groups(2).Name = 'Constant Wind'
      | sbobj.Groups(2).Signals(1).Name = 'Wind Speed'
      | sbobj.Groups(2).Signals(1).XData = [0 10 130]
      | sbobj.Groups(2).Signals(1).YData = [10 10 10]
      | sbobj.Groups(2).Signals(2).Name = 'Wind Direction'
      | sbobj.Groups(2).Signals(2).XData = [0 1 1 11 11 21 21 31 31 130]
      | sbobj.Groups(2).Signals(2).YData = [0 0 4 4 0 0 -4 -4 0 0]
      | sbobj.Groups(3).Name = 'High Wind Speed'
      | sbobj.Groups(3).Signals(1).Name = 'Wind Speed'
      | sbobj.Groups(3).Signals(1).XData = [0 10 60]
      | sbobj.Groups(3).Signals(1).YData = [10 9.9 25]
      | sbobj.Groups(3).Signals(2).Name = 'Wind Direction'
      | sbobj.Groups(3).Signals(2).XData = [0 1 11 21 31 60]
      | sbobj.Groups(3).Signals(2).YData = [0 0 4 0 -2.1 0]
      | sbobj.Groups(4).Name = 'Cut Out'
      | sbobj.Groups(4).Signals(1).Name = 'Wind Speed'
      | sbobj.Groups(4).Signals(1).XData = [0 5 25.1 28 60 75 121.8 130]
      | sbobj.Groups(4).Signals(1).YData = [10 10 8.7 7.85 9.65 2 2 2]
      | sbobj.Groups(4).Signals(2).Name = 'Wind Direction'
      | sbobj.Groups(4).Signals(2).XData = [0 1 1 11 11 21 21 31 31 130]
      | sbobj.Groups(4).Signals(2).YData = [0 0 4 4 0 0 -4 -4 0 0]
      | sbobj.Groups(5).Name = 'Start Stop'
      | sbobj.Groups(5).Signals(1).Name = 'Wind Speed'
      | sbobj.Groups(5).Signals(1).XData = [0 5 25 28 55 75 80 130]
      | sbobj.Groups(5).Signals(1).YData = [2 2 13 10 15 2 2 2]
      | sbobj.Groups(5).Signals(2).Name = 'Wind Direction'
      | sbobj.Groups(5).Signals(2).XData = [0 1 11 21 31 36.6 54.8 75 130]
      | sbobj.Groups(5).Signals(2).YData = [0 0 2.9 0.5 0.5 1.57171717172 -4 -4 -4]
      | sbobj.Groups(6).Name = 'Start Stop No Yaw'
      | sbobj.Groups(6).Signals(1).Name = 'Wind Speed'
      | sbobj.Groups(6).Signals(1).XData = [0 5 25 28 55 75 80 130]
      | sbobj.Groups(6).Signals(1).YData = [2 2 13 10 15 2 2 2]
      | sbobj.Groups(6).Signals(2).Name = 'Wind Direction'
      | sbobj.Groups(6).Signals(2).XData = [0 130]
      | sbobj.Groups(6).Signals(2).YData = [0 0]
      | sbobj.Groups(7).Name = 'Varying Wind'
      | sbobj.Groups(7).Signals(1).Name = 'Wind Speed'
      | sbobj.Groups(7).Signals(1).XData = [0 5 25 28 45 60.2 75 78.2 80 130]
      | sbobj.Groups(7).Signals(1).YData = [2 2 13 10 14.4 10.6 13.9 8 8 2]
      | sbobj.Groups(7).Signals(2).Name = 'Wind Direction'
      | sbobj.Groups(7).Signals(2).XData = [0 1 11 21 31 36.6 54.8 75 130]
      | sbobj.Groups(7).Signals(2).YData = [0 0 2.9 0.5 0.5 1.57171717172 -4 -4 -4]
  Wind Speed : Outport  Tag=STV Outport  VectorParamsAs1DForOutWhenUnconnected=off
  Wind Direction : Outport  Tag=STV Outport  Port=2  VectorParamsAs1DForOutWhenUnconnected=off
  wires:
  Demux/2 -> Wind Direction/1
  Demux/1 -> Wind Speed/1
  FromWs/1 -> Demux/1
